simulink model "Problem3a"  (R2026a)
settings: Solver=VariableStepAuto  StopTime=100
libraries: simulink x1

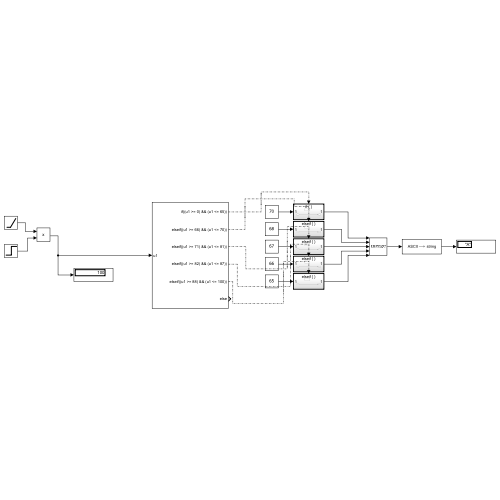
[thumbnail: Simulink's stored preview of the top-level diagram]
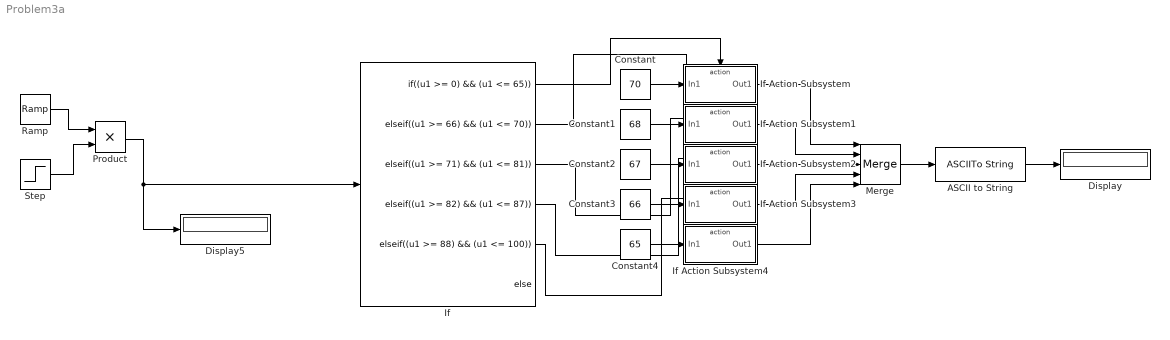
== system Problem3a ==
  ASCII to String : ASCIIToString
  Constant : Constant  Value=70  OutDataTypeStr=uint8
  Constant1 : Constant  Value=68  OutDataTypeStr=uint8
  Constant2 : Constant  Value=67  OutDataTypeStr=uint8
  Constant3 : Constant  Value=66  OutDataTypeStr=uint8
  Constant4 : Constant  Value=65  OutDataTypeStr=uint8
  Display : Display
  Display5 : Display
  If : If  IfExpression=(u1 >= 0) && (u1 <= 65)  ElseIfExpressions=(u1 >= 66) && (u1 <= 70),(u1 >= 71) && (u1 <= 81),(u1 >= 82) && (u1 <= 87),(u1 >= 88) && (u1 <= 100)
  If Action Subsystem : Subsystem  TreatAsAtomicUnit=on
  If Action Subsystem1 : Subsystem  TreatAsAtomicUnit=on
  If Action Subsystem2 : Subsystem  TreatAsAtomicUnit=on
  If Action Subsystem3 : Subsystem  TreatAsAtomicUnit=on
  If Action Subsystem4 : Subsystem  TreatAsAtomicUnit=on
  Merge : Merge  Inputs=5
  Product : Product
  Ramp : simulink/Sources/Ramp  slope=1  start=0  InitialOutput=0
  Step : Step  SampleTime=1
  wires:
  If/1 -> If Action Subsystem/Action
  Constant/1 -> If Action Subsystem/1(In1)
  If/2 -> If Action Subsystem1/Action
  Constant1/1 -> If Action Subsystem1/1(In1)
  If/3 -> If Action Subsystem2/Action
  Constant2/1 -> If Action Subsystem2/1(In1)
  Constant3/1 -> If Action Subsystem3/1(In1)
  If/4 -> If Action Subsystem3/Action
  Constant4/1 -> If Action Subsystem4/1(In1)
  If/5 -> If Action Subsystem4/Action
  Ramp/1 -> Product/1
  Step/1 -> Product/2
  Product/1 -> If/1, Display5/1
  If Action Subsystem/1(Out1) -> Merge/1
  If Action Subsystem1/1(Out1) -> Merge/2
  If Action Subsystem2/1(Out1) -> Merge/3
  If Action Subsystem3/1(Out1) -> Merge/4
  If Action Subsystem4/1(Out1) -> Merge/5
  ASCII to String/1 -> Display/1
  Merge/1 -> ASCII to String/1

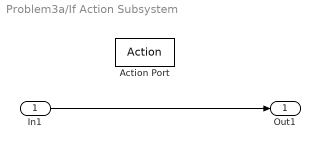
== system Problem3a/If Action Subsystem ==
  In1 : Inport
  Action Port : ActionPort  ActionPortLabel=if((u1 >= 0) && (u1 <= 65))
  Out1 : Outport
  wires:
  In1/1 -> Out1/1

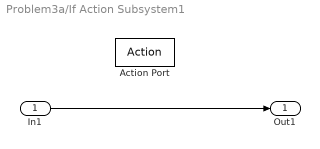
== system Problem3a/If Action Subsystem1 ==
  In1 : Inport
  Action Port : ActionPort  ActionPortLabel=elseif((u1 >= 66) && (u1 <= 70))
  Out1 : Outport
  wires:
  In1/1 -> Out1/1

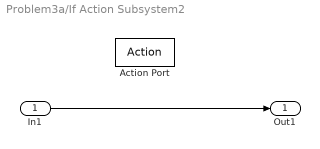
== system Problem3a/If Action Subsystem2 ==
  In1 : Inport
  Action Port : ActionPort  ActionPortLabel=elseif((u1 >= 71) && (u1 <= 81))
  Out1 : Outport
  wires:
  In1/1 -> Out1/1

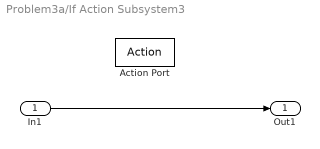
== system Problem3a/If Action Subsystem3 ==
  In1 : Inport
  Action Port : ActionPort  ActionPortLabel=elseif((u1 >= 82) && (u1 <= 87))
  Out1 : Outport
  wires:
  In1/1 -> Out1/1

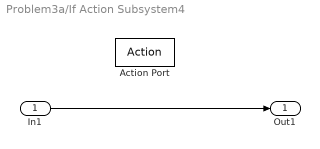
== system Problem3a/If Action Subsystem4 ==
  In1 : Inport
  Action Port : ActionPort  ActionPortLabel=elseif((u1 >= 88) && (u1 <= 100))
  Out1 : Outport
  wires:
  In1/1 -> Out1/1
